simulink subsystem "PowerSplitHEV_SpeedTracking_refsub"  (R2023a)
settings: Solver=VariableStepAuto  StartTime=0.0  StopTime=10.0  RelTol=1e-3
settings Model: Creator=isaacito  LastModifiedBy=isaacito
settings SolverCC: AlgebraicLoopSolver=TrustRegion
settings OptimizationCC: ReuseModelBlockBuffer=off
settings DebuggingCC: UnconnectedInputMsg=warning  UnconnectedOutputMsg=warning  UnconnectedLineMsg=warning
settings ModelReferenceCC: EnableRefExpFcnMdlSchedulingChecks=on
settings RTWCC: DLArmComputeVersion=19.05

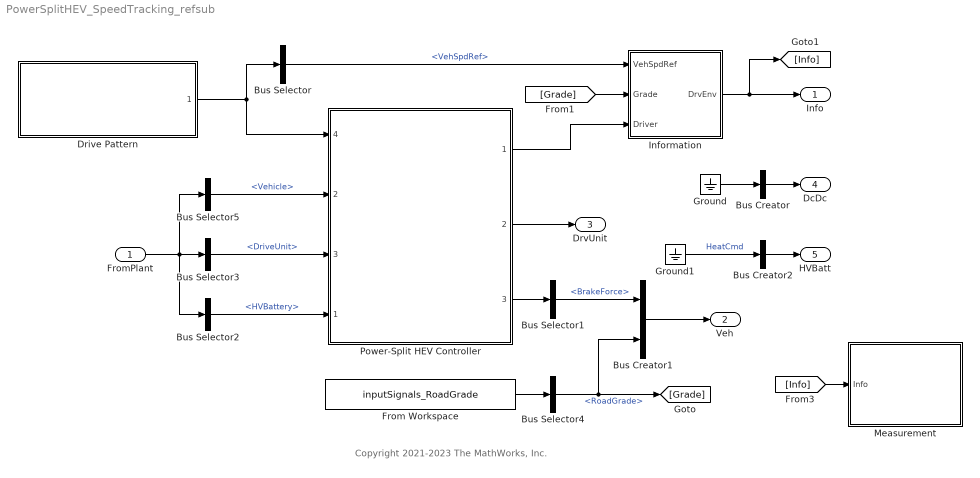
== system PowerSplitHEV_SpeedTracking_refsub ==
  note: Copyright 2021-2023 The MathWorks, Inc.
  FromPlant : Inport
  Bus Creator : BusCreator  Inputs=1
  Bus Creator1 : BusCreator  Inputs=2
  Bus Creator2 : BusCreator  Inputs=1
  Bus Selector : BusSelector  OutputSignals=VehSpdRef
  Bus Selector1 : BusSelector  OutputSignals=BrakeForce
  Bus Selector2 : BusSelector  OutputSignals=HVBattery
  Bus Selector3 : BusSelector  OutputSignals=DriveUnit
  Bus Selector4 : BusSelector  OutputSignals=RoadGrade
  Bus Selector5 : BusSelector  OutputSignals=Vehicle
  Drive Pattern : Subsystem  ReferencedSubsystem=DrivePattern_refsub
  From Workspace : FromWorkspace  VariableName=inputSignals_RoadGrade  OutDataTypeStr=Bus: inputBus_RoadGrade  Interpolate=off  OutputAfterFinalValue=Holding final value
      settings: AttributesFormatString=%<OutDataTypeStr>
  Ground : Ground
  Ground1 : Ground
  Information : Subsystem
  Measurement : Subsystem
  Power-Split HEV Controller : Subsystem  ReferencedSubsystem=HEVPowerSplitControl_refsub
      settings: PortSchema="{\"entries\":[{\"content\":{\"sides\":[{\"content\":{\"connectorIds\":[\"In4\",\"In2\",\"In3\",\"In1\"]},\"type\":\"ConnectorPlacement.EquallySpacedRectSide\",\"uuid\":\"5f20289c-1167-4559-b676-489e0a8e7832\"},{\"content\":{\"connectorIds\":[\"Out1\",\"Out2\",\"Out3\"],\"side\":\"RIGHT\"},\"type\":\"ConnectorPlacement.EquallySpacedRectSide\",\"uuid\":\"70a53654-f663-44c1-9472-875bd67166fb\"},{\"content\":{\"side\":\"TOP\"},\"type\":\"ConnectorPlacement.EquallySpacedRectSide\",\"uuid\":\"edc8af81-7bd0-4bb6-b9b6-6029ac3d73da\"},{\"content\":{\"side\":\"HIDDEN\"},\"type\":\"ConnectorPlacement.EquallySpacedRectSide\",\"uuid\":\"e774cd4c-fece-49f1-a4b4-be9c91194614\"}]},\"type\":\"ConnectorPlacement.EquallySpacedConnector\",\"uuid\":\"ed8c7061-c9d3-42a7-ab32-834a4768f508\"}],\"packageUris\":[\"http://schema.mathworks.com/mf0/Connector/R2020b\"],\"version\":\"1.0\"}"
  Info : Outport
  Veh : Outport  Port=2
  DrvUnit : Outport  Port=3
  DcDc : Outport  Port=4
  HVBatt : Outport  Port=5
  wires:
  From Workspace/1 -> Bus Selector4/1
  Power-Split HEV Controller/2 -> DrvUnit/1
  Drive Pattern/1 -> Bus Selector/1, Power-Split HEV Controller/4
  Bus Selector/1 -> Information/1(VehSpdRef)  "<VehSpdRef>"
  Power-Split HEV Controller/3 -> Bus Selector1/1
  Bus Selector1/1 -> Bus Creator1/1  "<BrakeForce>"
  Bus Creator1/1 -> Veh/1
  Bus Selector4/1 -> Bus Creator1/2, [Grade]  "<RoadGrade>"
  [Grade] -> Information/2(Grade)
  Information/1(DrvEnv) -> Info/1, [Info]
  FromPlant/1 -> Bus Selector2/1, Bus Selector3/1, Bus Selector5/1
  Bus Selector2/1 -> Power-Split HEV Controller/1  "<HVBattery>"
  Bus Selector3/1 -> Power-Split HEV Controller/3  "<DriveUnit>"
  Bus Selector5/1 -> Power-Split HEV Controller/2  "<Vehicle>"
  [Info] -> Measurement/1(Info)
  Power-Split HEV Controller/1 -> Information/3(Driver)
  Ground/1 -> Bus Creator/1
  Bus Creator/1 -> DcDc/1
  Bus Creator2/1 -> HVBatt/1
  Ground1/1 -> Bus Creator2/1  "HeatCmd"

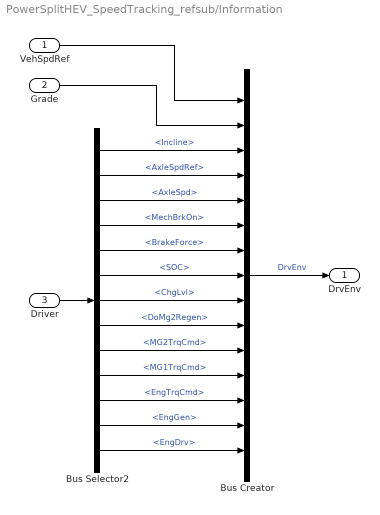
== system PowerSplitHEV_SpeedTracking_refsub/Information ==
  VehSpdRef : Inport
      settings: AttributesFormatString=%<Unit>
  Grade : Inport  Port=2
      settings: AttributesFormatString=%<Unit>
  Driver : Inport  Port=3
  Bus Creator : BusCreator  Inputs=15
  Bus Selector2 : BusSelector  OutputSignals=Incline,AxleSpdRef,AxleSpd,MechBrkOn,BrakeForce,SOC,ChgLvl,DoMg2Regen,MG2TrqCmd,MG1TrqCmd,EngTrqCmd,EngGen,EngDrv
  DrvEnv : Outport
  wires:
  Bus Selector2/1 -> Bus Creator/3  "<Incline>"
  Bus Selector2/13 -> Bus Creator/15  "<EngDrv>"
  Bus Selector2/12 -> Bus Creator/14  "<EngGen>"
  Bus Selector2/11 -> Bus Creator/13  "<EngTrqCmd>"
  Bus Selector2/10 -> Bus Creator/12  "<MG1TrqCmd>"
  Bus Selector2/9 -> Bus Creator/11  "<MG2TrqCmd>"
  Bus Selector2/8 -> Bus Creator/10  "<DoMg2Regen>"
  Bus Selector2/7 -> Bus Creator/9  "<ChgLvl>"
  Bus Selector2/6 -> Bus Creator/8  "<SOC>"
  Bus Selector2/5 -> Bus Creator/7  "<BrakeForce>"
  Bus Selector2/4 -> Bus Creator/6  "<MechBrkOn>"
  Driver/1 -> Bus Selector2/1
  Grade/1 -> Bus Creator/2
  VehSpdRef/1 -> Bus Creator/1
  Bus Selector2/2 -> Bus Creator/4  "<AxleSpdRef>"
  Bus Creator/1 -> DrvEnv/1  "DrvEnv"
  Bus Selector2/3 -> Bus Creator/5  "<AxleSpd>"

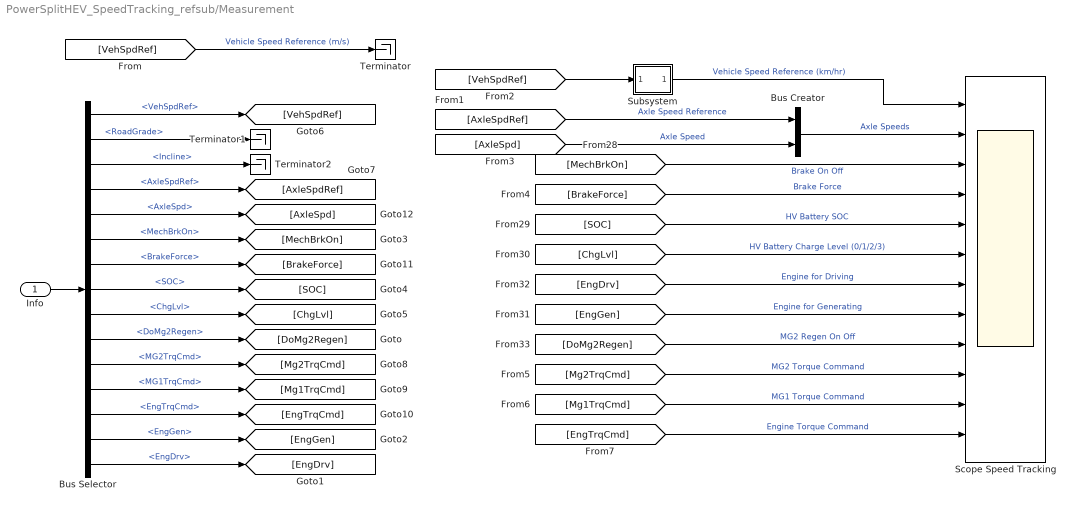
== system PowerSplitHEV_SpeedTracking_refsub/Measurement ==
  Info : Inport
  Bus Creator : BusCreator  Inputs=2
  Bus Selector : BusSelector  OutputSignals=VehSpdRef,RoadGrade,Incline,AxleSpdRef,AxleSpd,MechBrkOn,BrakeForce,SOC,ChgLvl,DoMg2Regen,MG2TrqCmd,MG1TrqCmd,EngTrqCmd,EngGen,EngDrv
  Scope Speed Tracking : Scope  NumInputPorts=12
  Subsystem : Subsystem
  Terminator : Terminator
  Terminator1 : Terminator
  Terminator2 : Terminator
  wires:
  [EngTrqCmd] -> Scope Speed Tracking/12  "Engine Torque Command"
  [Mg1TrqCmd] -> Scope Speed Tracking/11  "MG1 Torque Command"
  [Mg2TrqCmd] -> Scope Speed Tracking/10  "MG2 Torque Command"
  [DoMg2Regen] -> Scope Speed Tracking/9  "MG2 Regen On Off"
  [EngGen] -> Scope Speed Tracking/8  "Engine for Generating"
  [EngDrv] -> Scope Speed Tracking/7  "Engine for Driving"
  [ChgLvl] -> Scope Speed Tracking/6  "HV Battery Charge Level (0/1/2/3)"
  [SOC] -> Scope Speed Tracking/5  "HV Battery SOC"
  [BrakeForce] -> Scope Speed Tracking/4  "Brake Force"
  [MechBrkOn] -> Scope Speed Tracking/3  "Brake On Off"
  Bus Creator/1 -> Scope Speed Tracking/2  "Axle Speeds"
  Subsystem/1(spd) -> Scope Speed Tracking/1  "Vehicle Speed Reference (km/hr)"
  [VehSpdRef] -> Terminator/1  "Vehicle Speed Reference (m/s)"
  [VehSpdRef] -> Subsystem/1(In1)
  [AxleSpd] -> Bus Creator/2  "Axle Speed"
  [AxleSpdRef] -> Bus Creator/1  "Axle Speed Reference"
  Bus Selector/15 -> [EngDrv]  "<EngDrv>"
  Bus Selector/14 -> [EngGen]  "<EngGen>"
  Bus Selector/13 -> [EngTrqCmd]  "<EngTrqCmd>"
  Bus Selector/12 -> [Mg1TrqCmd]  "<MG1TrqCmd>"
  Bus Selector/11 -> [Mg2TrqCmd]  "<MG2TrqCmd>"
  Bus Selector/10 -> [DoMg2Regen]  "<DoMg2Regen>"
  Bus Selector/9 -> [ChgLvl]  "<ChgLvl>"
  Bus Selector/8 -> [SOC]  "<SOC>"
  Bus Selector/7 -> [BrakeForce]  "<BrakeForce>"
  Bus Selector/6 -> [MechBrkOn]  "<MechBrkOn>"
  Bus Selector/5 -> [AxleSpd]  "<AxleSpd>"
  Bus Selector/4 -> [AxleSpdRef]  "<AxleSpdRef>"
  Bus Selector/3 -> Terminator2/1  "<Incline>"
  Bus Selector/2 -> Terminator1/1  "<RoadGrade>"
  Bus Selector/1 -> [VehSpdRef]  "<VehSpdRef>"
  Info/1 -> Bus Selector/1

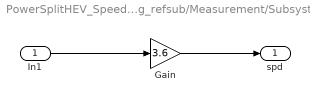
== system PowerSplitHEV_SpeedTracking_refsub/Measurement/Subsystem ==
  In1 : Inport  Unit=m/s
  Gain : Gain  Gain=3.6
  spd : Outport  Unit=km/hr
  wires:
  Gain/1 -> spd/1
  In1/1 -> Gain/1
